simulink model "FMS"  (R2018b)
settings: configuration reference "fms_config" (kept outside this file)
values from neighbouring files (symbols this model uses):
  FMS_EXPORT = Simulink.Parameter(FMS_EXPORT_VALUE)    [fms_model_init.m]
  FMS_PARAM = Simulink.Parameter(FMS_PARAM_VALUE)    [fms_model_init.m]
undefined symbols (not defined in the file or in its folder): actuator_cmd, ax_cmd, ay_cmd, az_cmd, cmd_mask, ControlMode, ctrl_mode, DiscIntNeverNeededParam, ext_state, FMS_Cmd, FMS_CONST, home, mode, p_cmd, phi_cmd, PilotMode, psi_rate_cmd, q_cmd, r_cmd, reset, state, status, theta_cmd, throttle_cmd, timestamp, u_cmd, v_cmd, VehicleState, VehicleStatus, VTOLState, w_cmd, wp_consume, wp_current
libraries: simulink x141, FMT_Model_Lib x120, hdlsllib x13
(part 11 of 12)

== matlab function FMS/FMS Commander/Commander/Arm/MC_Mode/Auto/Mission/Mission_SubSystem/Velocity Commander/L1 Reference WP/SearchL1RefWP ==
  data: P1 input; P output; P2 input; P3 input; L1 input; u output
% Find reference waypoint (L1RefWP) on the line segment P1P2 which has 
% L1 distance from vehicle position (P3).
%
% The idea is to calculate the intersection point of a circle with L1 radius
% with the line segment P1P2.
%
% Define P = P1 + u * (P2 - P1), where P is the intersection point.
% Goal is calculating the u, where the valid u is between [0, 1].
%
% Input:
%   P1: start point of segment line
%   P2: start point of segment line
%   P3: circle center point, also is known as the vehicle position
%   L1: the L1 distance
% Output:
%   P: L1 reference waypoint
%   u: scale factor (valid between 0 and 1), -1 means no intersection.
function [P, u] = SearchL1RefWP(P1, P2, P3, L1)

% P1 = (x1, y1), P2 = (x2, y2), P3 = (x3, y3)
x1 = P1(1);
y1 = P1(2);
x2 = P2(1);
y2 = P2(2);
x3 = P3(1);
y3 = P3(2);

% The P is on circle and line segment, which yields:
A = (x2 - x1)^2 + (y2 - y1)^2;
B = 2 * ((x2 - x1)*(x1 - x3) + (y2 - y1)*(y1 - y3));
C = x3^2 + y3^2 + x1^2 + y1^2 - 2*(x3*x1 + y3*y1) - L1^2;
% Check root existence confition if B^2 - 4*A*C >= 0
D = B^2 - 4*A*C;
u = single(-1);
P = single([0 0]);

if D > 0
    % D>0 means we have 2 difference roots, % root is valid only if u is in range of [0, 1]
    u1 = (-B + sqrt(D)) / (2*A);
    u2 = (-B - sqrt(D)) / (2*A);
    
    if (u1>=0 && u1<=1) && (u2>=0 && u2<=1)
        % have 2 valid roots, select the one which is closer to P2 (target point)
        if u1 > u2
            u = u1; 
        else
            u = u2;
        end
    elseif (u1>=0 && u1<=1)
        % only 1 root valid, select it
        u = u1;
    elseif (u2>=0 && u2<=1)
        % only 1 root valid, select it
        u = u2;
    else
        % no valid root, which means no intersection point founded.
        return;
    end
elseif D == 0
    % D=0 means only 1 single root
    u1 = -B / (2*A);
    if (u1>=0 && u1<=1)
        % valid root, select it
        u = u1;
    else
        % no valid root, which means no intersection point founded.
        return;
    end
else
    % no valid root, which means no intersection point founded.
    return;
end

% calculate the L1 reference waypoint (P) coordinate
P(1) = x1 + u*(x2 - x1);
P(2) = y1 + u*(y2 - y1);

== stateflow chart FMS/FMS Commander/Commander/Arm/FW_Mode/Assist/Altitude/Altitude Command/Detect Movement/Motion Status ==
  state Hold
    entry:
    state=MotionState.Hold;
  state Move
    entry:
    state=MotionState.Move;
  state Brake
    entry:
    state=MotionState.Brake;
  (default) -> Move
  Hold -> Move : [motion_req==1]
  Move -> Brake : [motion_req==0]
  Brake -> Move [order 2] : [motion_req==1]
  Brake -> Hold [order 1] : [speed<=0.15 || after(1.5, sec)]
  data: state output Enum: MotionState; motion_req input; speed input

== stateflow chart FMS/FMS State Machine ==
  state Command_Listener [parallel]
    settings: executionOrder=1
    state Send
      entry:
      % Send command
      M.data=save_cmd;
      send(M);
    state Listen
    state Check
      entry:
      valid_cmd = CheckCmdValid(save_cmd, mode, INS_Out.flag);
    (default) -> Command_Listener.Listen
    Command_Listener.Send -> Command_Listener.Listen
    Command_Listener.Listen -> Command_Listener.Check : [hasChanged(cmd) && ...
        | cmd ~= FMS_Cmd.None]{save_cmd = cmd;}
    Command_Listener.Check -> Command_Listener.Listen [order 2]
    Command_Listener.Check -> Command_Listener.Send [order 1] : [valid_cmd == true]
  state Vehicle [parallel]
    du:
    % if mission data updated, reset waypoint index
    if hasChanged(mission_timestamp)
    wp_consume = 0;
    wp_index = 1;
    need_forwardtrans = 0;
    end
    settings: executionOrder=6
    state moved = StickMoved(stick_val,pilot_cmd) [function]
    state sp_takeoff = PrepTakeoff(xy_R) [function]
    state radius = AcceptRadius(state) [function]
    state err = HeadingErr(psi_cmd, psi_est) [function]
    state angle = WaypointAngle(start, end) [function]
    state Arm
      en:
      status = VehicleStatus.Arm;
      state SubMode
        en:
        % save enter stick value
        stick_val = [Pilot_Cmd.stick_yaw; Pilot_Cmd.stick_throttle; Pilot_Cmd.stick_roll; Pilot_Cmd.stick_pitch];
        state Return
          en:
          Cmd_In.cur_waypoint = [INS_Out.x_R; INS_Out.y_R; INS_Out.h_R];
          Cmd_In.sp_waypoint = [home(1); home(2); INS_Out.h_R]
          state Align
            en:
            Cmd_In.set_yaw = WaypointAngle(Cmd_In.cur_waypoint, Cmd_In.sp_waypoint);
            state = VehicleState.Hold;
          state Wait
          state ForwardTrans
            en:
            VTOL_M.data=VTOLMode.Fixwing;
            send(VTOL_M);
          state Execute
            en:
            state = VehicleState.Return;
          (default) -> (junction 1189)
          (junction 1189) -> Vehicle.Arm.SubMode.Return.Align [order 1] : [norm([INS_Out.x_R,INS_Out.y_R] - [home(1),home(2)]) ...
              | > 2 * AcceptRadius(VTOLState.Fixwing) && vtol_state == VTOLState.Multicopter]
          (junction 1189) -> Vehicle.Arm.SubMode.Return.Execute [order 2]
          Vehicle.Arm.SubMode.Return.Align -> Vehicle.Arm.SubMode.Return.Wait : [abs(HeadingErr(Cmd_In.set_yaw, INS_Out.psi)) <= 5/180*pi]
          Vehicle.Arm.SubMode.Return.Wait -> Vehicle.Arm.SubMode.Return.ForwardTrans : after(3, sec)
          Vehicle.Arm.SubMode.Return.ForwardTrans -> Vehicle.Arm.SubMode.Return.Execute : [vtol_state == VTOLState.ForwardTrans || ...
              | vtol_state == VTOLState.Fixwing]
        state Land
          en:
          state = VehicleState.Land;
          state MC_Land
            en:
            state = VehicleState.Land;
          state VTOL_Land
            state BackTrans
              en:
              % send BackTrans command
              VTOL_M.data=VTOLMode.Multicopter;
              send(VTOL_M);
            state Return
              en:
              Cmd_In.cur_waypoint = [INS_Out.x_R; INS_Out.y_R; INS_Out.h_R];
              Cmd_In.sp_waypoint(3) = INS_Out.h_R;
              state = VehicleState.Return;
            (default) -> Vehicle.Arm.SubMode.Land.VTOL_Land.BackTrans
            Vehicle.Arm.SubMode.Land.VTOL_Land.BackTrans -> Vehicle.Arm.SubMode.Land.VTOL_Land.Return : [vtol_state == VTOLState.Multicopter]
          Vehicle.Arm.SubMode.Land.VTOL_Land.Return -> MC_Land : [norm([INS_Out.x_R,INS_Out.y_R]-Cmd_In.sp_waypoint(1:2)') ...
              | <= AcceptRadius(vtol_state)]
          (default) -> (junction 1157)
          (junction 1157) -> Vehicle.Arm.SubMode.Land.VTOL_Land [order 2]
          (junction 1157) -> MC_Land [order 1] : [vtol_state == VTOLState.Multicopter]
        state Takeoff
          en:
          state = VehicleState.Takeoff;
        state Hold
          state BackTrans
            en:
            % If enter hold from mission, when back to mission we recover the previous vtol mode
            if state == VehicleState.Mission && ...
            (vtol_state == VTOLState.Fixwing || vtol_state == VTOLState.ForwardTrans)
            need_forwardtrans = 1;
            end
            % send BackTrans command
            VTOL_M.data=VTOLMode.Multicopter;
            send(VTOL_M);
          state Loiter
            en:
            Cmd_In.sp_waypoint = [INS_Out.x_R; INS_Out.y_R; INS_Out.h_R];
            Cmd_In.set_yaw = single(-1);
            state = VehicleState.Hold;
          (default) -> (junction 1226)
          (junction 1226) -> Vehicle.Arm.SubMode.Hold.BackTrans [order 2]
          (junction 1226) -> Vehicle.Arm.SubMode.Hold.Loiter [order 1] : [vtol_state == VTOLState.Multicopter]
          Vehicle.Arm.SubMode.Hold.BackTrans -> Vehicle.Arm.SubMode.Hold.Loiter : [vtol_state == VTOLState.Multicopter]
        Vehicle.Arm.SubMode.Takeoff -> (junction 612) : [INS_Out.h_R >= Cmd_In.sp_waypoint(3)]
        (junction 612) -> Vehicle.Arm.SubMode.Hold [order 2]
        SubMode -> Vehicle.Arm.SubMode.Hold [order 1] : M[M.data==FMS_Cmd.Pause]
        Vehicle.Arm.SubMode.Return.Execute -> Vehicle.Arm.SubMode.Land : [norm([INS_Out.x_R;INS_Out.y_R] - Cmd_In.sp_waypoint(1:2)) <= ...
            |  AcceptRadius(vtol_state)]{
            | Cmd_In.sp_waypoint = [home(1); home(2); 0]}
      state Auto
        state Offboard
          state Loiter
            en:
            state = VehicleState.Hold;
          state Run
            en:
            state = VehicleState.Offboard;
          (default) -> (junction 958)
          (junction 958) -> Vehicle.Arm.Auto.Offboard.Loiter [order 2]
          (junction 958) -> Run [order 1] : [auto_cmd_valid == 1]
          Run -> Vehicle.Arm.Auto.Offboard.Loiter : [auto_cmd_valid == 0]
          Vehicle.Arm.Auto.Offboard.Loiter -> Run : [auto_cmd_valid == 1]
        state Mission
          en:
          % Reference location of latitude and longitude, specified as an m-by-2 array, in degrees
          llo = [INS_Out.lat_0, INS_Out.lon_0] * (180/pi);
          % Set setpoint waypoint to current position
          Cmd_In.sp_waypoint = [INS_Out.x_R; INS_Out.y_R; INS_Out.h_R];
          Cmd_In.set_speed = 0;
          state pos = LLA2FLAT(lla,llo,href,psio) [function]
          state Loiter
            en:
            Cmd_In.sp_waypoint = [INS_Out.x_R; INS_Out.y_R; INS_Out.h_R];
            Cmd_In.set_yaw = single(-1);
            state = VehicleState.Hold;
          state NextWP
            en:
            if wp_index <= Mission_Data.valid_items
            nav_cmd = Mission_Data.command(wp_index);
            else
            nav_cmd = uint16(NAV_Cmd.None);
            % updated consumed waypoints
            wp_consume = wp_index - 1;
            end
          state Takeoff
            state Takeoff
              en:
              % Geodetic coordinates (latitude, longitude, and altitude), specified as an m-by-3 array in [degrees degrees meters]
              % Altitude add home(3) here because the altitude when takeoff could be non-zero
              lla = [double(Mission_Data.x(wp_index))*1e-7, double(Mission_Data.y(wp_index))*1e-7, double(-(Mission_Data.z(wp_index) + home(3)))];
              % set takeoff setpoint
              Cmd_In.sp_waypoint = LLA2FLAT(lla, llo, 0, 0);
              % enter takeoff state
              state = VehicleState.Takeoff;
            state Waypoint
              en:
              % set current waypoint to previous setpoint waypoint
              Cmd_In.cur_waypoint  = [INS_Out.x_R; INS_Out.y_R; INS_Out.h_R];
              state = VehicleState.Mission;
            (default) -> Vehicle.Arm.Auto.Mission.Takeoff.Takeoff
            Vehicle.Arm.Auto.Mission.Takeoff.Takeoff -> (junction 1270) : [INS_Out.h_R >= Cmd_In.sp_waypoint(3)]
            (junction 1270) -> (junction 1272) [order 2]
            (junction 1270) -> Vehicle.Arm.Auto.Mission.Takeoff.Waypoint [order 1] : [norm([INS_Out.x_R;INS_Out.y_R] - Cmd_In.sp_waypoint(1:2)) > ...
                |  AcceptRadius(vtol_state)]
            Vehicle.Arm.Auto.Mission.Takeoff.Waypoint -> (junction 1272) : [norm([INS_Out.x_R;INS_Out.y_R] - Cmd_In.sp_waypoint(1:2)) <= ...
                |  AcceptRadius(vtol_state)]
          state Waypoint
            en:
            % Geodetic coordinates (latitude, longitude, and altitude), specified as an m-by-3 array in [degrees degrees meters]
            % Altitude add home(3) here because the altitude when takeoff could be non-zero
            lla = [double(Mission_Data.x(wp_index))*1e-7, double(Mission_Data.y(wp_index))*1e-7, double(-(Mission_Data.z(wp_index) + home(3)))];
            % set current waypoint to previous setpoint waypoint
            Cmd_In.cur_waypoint = Cmd_In.sp_waypoint;
            % target waypoint
            Cmd_In.sp_waypoint = LLA2FLAT(lla, llo, 0, 0);
            state Align
              en:
              Cmd_In.set_yaw = WaypointAngle(Cmd_In.cur_waypoint, Cmd_In.sp_waypoint);
              state = VehicleState.Hold;
            state Hold
              en:
              Cmd_In.set_yaw = single(-1);
              state = VehicleState.Hold;
            state Wait
            state Execute
              en:
              if need_forwardtrans
              need_forwardtrans = 0;
              end
              state = VehicleState.Mission;
            state ForwardTrans
              en:
              VTOL_M.data=VTOLMode.Fixwing;
              send(VTOL_M);
            (default) -> (junction 1112)
            (junction 1112) -> Vehicle.Arm.Auto.Mission.Waypoint.Align [order 1] : [need_forwardtrans && vtol_state == VTOLState.Multicopter]
            (junction 1112) -> Vehicle.Arm.Auto.Mission.Waypoint.Execute [order 2]
            Vehicle.Arm.Auto.Mission.Waypoint.Hold -> (junction 1323) : after(Mission_Data.param1(wp_index),sec)
            Vehicle.Arm.Auto.Mission.Waypoint.Align -> Vehicle.Arm.Auto.Mission.Waypoint.Wait : [abs(HeadingErr(Cmd_In.set_yaw, INS_Out.psi)) <= 5/180*pi]
            (junction 1320) -> (junction 1323) [order 2]
            (junction 1320) -> Vehicle.Arm.Auto.Mission.Waypoint.Hold [order 1] : [Mission_Data.param1(wp_index) > 0]
            Vehicle.Arm.Auto.Mission.Waypoint.Wait -> Vehicle.Arm.Auto.Mission.Waypoint.ForwardTrans : after(2, sec)
            Vehicle.Arm.Auto.Mission.Waypoint.ForwardTrans -> Vehicle.Arm.Auto.Mission.Waypoint.Execute : [vtol_state == VTOLState.ForwardTrans || ...
                | vtol_state == VTOLState.Fixwing]
            Vehicle.Arm.Auto.Mission.Waypoint.Execute -> (junction 1320) : [norm([INS_Out.x_R;INS_Out.y_R] - Cmd_In.sp_waypoint(1:2)) <= ...
                |  AcceptRadius(vtol_state)]
          state Disarming
          state Transition
            en:
            if Mission_Data.param1(wp_index) == 3
            VTOL_M.data=VTOLMode.Multicopter;
            send(VTOL_M);
            elseif Mission_Data.param1(wp_index) == 4
            need_forwardtrans = 1;
            end
          state WaitBackTransCplt
          state Return
            en:
            % set return target pos to home
            Cmd_In.cur_waypoint = Cmd_In.sp_waypoint;
            Cmd_In.sp_waypoint = [home(1); home(2); INS_Out.h_R];
            state Align
              en:
              Cmd_In.set_yaw = WaypointAngle(Cmd_In.cur_waypoint, Cmd_In.sp_waypoint);
              state = VehicleState.Hold;
            state Wait
            state ForwardTrans
              en:
              VTOL_M.data=VTOLMode.Fixwing;
              send(VTOL_M);
            state Execute
              en:
              if need_forwardtrans
              need_forwardtrans = 0;
              end
              state = VehicleState.Return;
            (default) -> (junction 1172)
            (junction 1172) -> Vehicle.Arm.Auto.Mission.Return.Align [order 1] : [need_forwardtrans && vtol_state == VTOLState.Multicopter]
            (junction 1172) -> Vehicle.Arm.Auto.Mission.Return.Execute [order 2]
            Vehicle.Arm.Auto.Mission.Return.Align -> Vehicle.Arm.Auto.Mission.Return.Wait : [abs(HeadingErr(Cmd_In.set_yaw, INS_Out.psi)) <= 5/180*pi]
            Vehicle.Arm.Auto.Mission.Return.Wait -> Vehicle.Arm.Auto.Mission.Return.ForwardTrans : after(2, sec)
            Vehicle.Arm.Auto.Mission.Return.ForwardTrans -> Vehicle.Arm.Auto.Mission.Return.Execute : [vtol_state == VTOLState.ForwardTrans || ...
                | vtol_state == VTOLState.Fixwing]
          state VTOL_Land
            state Waypoint
              en:
              % Geodetic coordinates (latitude, longitude, and altitude), specified as an m-by-3 array in [degrees degrees meters]
              % Altitude add home(3) here because the altitude when takeoff could be non-zero
              lla = [double(Mission_Data.x(wp_index))*1e-7, double(Mission_Data.y(wp_index))*1e-7, double(-(Mission_Data.z(wp_index) + home(3)))];
              % set current waypoint to previous setpoint waypoint
              Cmd_In.cur_waypoint = Cmd_In.sp_waypoint;
              % target waypoint
              Cmd_In.sp_waypoint = LLA2FLAT(lla, llo, 0, 0);
              state Align
                en:
                Cmd_In.set_yaw = WaypointAngle(Cmd_In.cur_waypoint, Cmd_In.sp_waypoint);
                state = VehicleState.Hold;
              state Wait
              state ForwardTrans
                en:
                VTOL_M.data=VTOLMode.Fixwing;
                send(VTOL_M);
              state Execute
                en:
                if need_forwardtrans
                need_forwardtrans = 0;
                end
                state = VehicleState.Mission;
              (default) -> (junction 1282)
              (junction 1282) -> Vehicle.Arm.Auto.Mission.VTOL_Land.Waypoint.Align [order 1] : [need_forwardtrans && vtol_state == VTOLState.Multicopter]
              (junction 1282) -> Vehicle.Arm.Auto.Mission.VTOL_Land.Waypoint.Execute [order 2]
              Vehicle.Arm.Auto.Mission.VTOL_Land.Waypoint.Align -> Vehicle.Arm.Auto.Mission.VTOL_Land.Waypoint.Wait : [abs(HeadingErr(Cmd_In.set_yaw, INS_Out.psi)) <= 5/180*pi]
              Vehicle.Arm.Auto.Mission.VTOL_Land.Waypoint.Wait -> Vehicle.Arm.Auto.Mission.VTOL_Land.Waypoint.ForwardTrans : after(2, sec)
              Vehicle.Arm.Auto.Mission.VTOL_Land.Waypoint.ForwardTrans -> Vehicle.Arm.Auto.Mission.VTOL_Land.Waypoint.Execute : [vtol_state == VTOLState.ForwardTrans || ...
                  | vtol_state == VTOLState.Fixwing]
            state BackTrans
              en:
              % send BackTrans command
              VTOL_M.data=VTOLMode.Multicopter;
              send(VTOL_M);
            state Return
              en:
              Cmd_In.cur_waypoint = [INS_Out.x_R; INS_Out.y_R; INS_Out.h_R];
              % Return to land position
              if nav_cmd == NAV_Cmd.VTOL_Land || nav_cmd == NAV_Cmd.Land
              lla = [double(Mission_Data.x(wp_index))*1e-7, double(Mission_Data.y(wp_index))*1e-7, 0];
              flat = LLA2FLAT(lla, llo, 0, 0);
              Cmd_In.sp_waypoint = [flat(1); flat(2); INS_Out.h_R];
              else
              Cmd_In.sp_waypoint = [home(1); home(2); INS_Out.h_R]
              end
              state = VehicleState.Return;
            state Land
              en:
              if nav_cmd == NAV_Cmd.Land || nav_cmd == NAV_Cmd.VTOL_Land
              lla = [double(Mission_Data.x(wp_index))*1e-7, double(Mission_Data.y(wp_index))*1e-7, 0];
              Cmd_In.sp_waypoint = LLA2FLAT(lla, llo, 0, 0);
              else
              Cmd_In.sp_waypoint = [home(1); home(2); 0]
              end
              state = VehicleState.Land;
            (default) -> (junction 1278)
            (junction 1278) -> (junction 1305) [order 2]
            (junction 1278) -> Vehicle.Arm.Auto.Mission.VTOL_Land.Waypoint [order 1] : [nav_cmd == NAV_Cmd.Land || ...
                | nav_cmd == NAV_Cmd.VTOL_Land]
            (junction 1305) -> (junction 1300)
            (junction 1300) -> Vehicle.Arm.Auto.Mission.VTOL_Land.BackTrans [order 2]
            (junction 1300) -> Vehicle.Arm.Auto.Mission.VTOL_Land.Land [order 1] : [vtol_state == VTOLState.Multicopter]
            Vehicle.Arm.Auto.Mission.VTOL_Land.Waypoint.Execute -> (junction 1300) : [norm([INS_Out.x_R;INS_Out.y_R] - Cmd_In.sp_waypoint(1:2)) <= ...
                |  AcceptRadius(vtol_state)]
            Vehicle.Arm.Auto.Mission.VTOL_Land.BackTrans -> Vehicle.Arm.Auto.Mission.VTOL_Land.Return : [vtol_state == VTOLState.Multicopter]
            Vehicle.Arm.Auto.Mission.VTOL_Land.Return -> Vehicle.Arm.Auto.Mission.VTOL_Land.Land : [norm([INS_Out.x_R,INS_Out.y_R]-Cmd_In.sp_waypoint(1:2)') ...
                | <= AcceptRadius(vtol_state)]
          Mission -> NextWP : [hasChanged(mission_timestamp)]
              | {Cmd_In.set_speed = 0}
          Vehicle.Arm.Auto.Mission.VTOL_Land.Land -> (junction 1316) : [duration(on_ground) >= 2]
          (junction 1323) -> (junction 879)
          (junction 1272) -> (junction 873)
          (junction 908) -> (junction 910) : {wp_index = wp_index + 1;}
          (junction 910) -> NextWP
          (junction 873) -> (junction 908)
          (default) -> NextWP
          NextWP -> Vehicle.Arm.Auto.Mission.Takeoff [order 1] : [nav_cmd == NAV_Cmd.Takeoff && ...
              | vtol_state == VTOLState.Multicopter]
          (junction 879) -> (junction 873)
          (junction 917) -> Vehicle.Arm.Auto.Mission.Loiter [order 2]
          (junction 1119) -> Vehicle.Arm.Auto.Mission.Takeoff
          NextWP -> (junction 1119) [order 2] : [nav_cmd == NAV_Cmd.VTOL_Takeoff && ...
              | vtol_state == VTOLState.Multicopter]{need_forwardtrans = 1;}
          NextWP -> (junction 917) [order 8]
          (junction 917) -> Disarming [order 1] : [on_ground]
          NextWP -> Vehicle.Arm.Auto.Mission.Waypoint [order 3] : [nav_cmd == NAV_Cmd.Waypoint]
          (junction 1077) -> (junction 879)
          Vehicle.Arm.Auto.Mission.Return.Execute -> Vehicle.Arm.Auto.Mission.VTOL_Land : [norm([INS_Out.x_R;INS_Out.y_R] - Cmd_In.sp_waypoint(1:2)) <= ...
              |  AcceptRadius(vtol_state)]
          Transition -> (junction 1077) [order 2]
          NextWP -> Transition [order 4] : [nav_cmd == NAV_Cmd.VTOL_Transition]
          (junction 1076) -> (junction 1077)
          Transition -> WaitBackTransCplt [order 1] : [Mission_Data.param1(wp_index) == 3]
          NextWP -> (junction 1314) [order 5] : [nav_cmd == NAV_Cmd.SetSpeed]{
              | Cmd_In.set_speed = Mission_Data.param2(wp_index)}
          (junction 1314) -> (junction 1316)
          NextWP -> Vehicle.Arm.Auto.Mission.Return [order 7] : [nav_cmd == NAV_Cmd.Return]
          NextWP -> Vehicle.Arm.Auto.Mission.VTOL_Land [order 6] : [nav_cmd == NAV_Cmd.Land || ...
              | nav_cmd == NAV_Cmd.VTOL_Land]
          WaitBackTransCplt -> (junction 1076) : [vtol_state == VTOLState.Multicopter]
          (junction 915) -> (junction 1076)
          (junction 1316) -> (junction 915)
        state InvalidAutoMode
        (default) -> (junction 43)
        (junction 43) -> Offboard [order 1] : [mode == PilotMode.Offboard]
        (junction 43) -> (junction 134) [order 2]
        (junction 134) -> Mission [order 1] : [mode == PilotMode.Mission]
        (junction 134) -> InvalidAutoMode [order 2]
        Disarming -> (junction 370)
        InvalidAutoMode -> (junction 370)
      state Assist
        state InvalidAssistMode
        state Acro
          en:
          state = VehicleState.Acro;
        state Stabilize
          en:
          state = VehicleState.Stabilize;
        state Altitude
          en:
          state = VehicleState.Altitude;
        state Position
          en:
          state = VehicleState.Position;
        (default) -> (junction 354)
        (junction 354) -> (junction 190) [order 2]
        (junction 190) -> (junction 193) [order 2]
        (junction 193) -> (junction 196) [order 2]
        (junction 196) -> InvalidAssistMode [order 2]
        (junction 354) -> Acro [order 1] : [mode == PilotMode.Acro]
        (junction 190) -> Stabilize [order 1] : [mode == PilotMode.Stabilize]
        (junction 193) -> Altitude [order 1] : [mode == PilotMode.Altitude]
        (junction 196) -> Position [order 1] : [mode == PilotMode.Position]
      state Manual
        state InValidManualMode
        state Manual
          en:
          state = VehicleState.Manual;
        (default) -> (junction 410)
        (junction 410) -> InValidManualMode [order 2]
        (junction 410) -> Vehicle.Arm.Manual.Manual [order 1] : [mode == PilotMode.Manual]
      state InvalidArmMode
      Vehicle.Arm -> Vehicle.Arm.SubMode.Land [order 2] : M[M.data==FMS_Cmd.Land]
          | {Cmd_In.sp_waypoint = [INS_Out.x_R; INS_Out.y_R; 0]}
      Vehicle.Arm -> Vehicle.Arm.SubMode.Return [order 3] : M[M.data==FMS_Cmd.Return]
      Vehicle.Arm.SubMode.Hold -> Vehicle.Arm : M[M.data==FMS_Cmd.Continue ...
          | && mode ~= PilotMode.None]
      (junction 612) -> (junction 117) [order 1] : [mode ~= PilotMode.None]
      Auto -> Vehicle.Arm.SubMode.Hold : M[M.data==FMS_Cmd.Pause]
      SubMode -> (junction 117) [order 1] : [(StickMoved(stick_val, Pilot_Cmd) || ...
          | bitand(INS_Out.flag, 212) ~= 212) && ...
          | (getArmMode(mode) == 1 || getArmMode(mode) == 2)]
      Vehicle.Arm -> (junction 117) [order 1] : [hasChanged(mode) && ...
          | mode ~= PilotMode.None]
      (junction 117) -> Auto [order 1] : [getArmMode(mode) == 3]
      (default) -> (junction 117)
      (junction 117) -> (junction 140) [order 2]
      (junction 140) -> Assist [order 1] : [getArmMode(mode)  == 2]
      (junction 140) -> (junction 240) [order 2]
      (junction 240) -> Vehicle.Arm.Manual [order 1] : [getArmMode(mode)  == 1]
      (junction 240) -> InvalidArmMode [order 2]
    state Standby
      en:
      % check if mission takeoff is valid
      if mode==PilotMode.Mission
      if wp_index <= Mission_Data.valid_items > 0 && ...
      (Mission_Data.command(wp_index)==NAV_Cmd.Takeoff || ...
      Mission_Data.command(wp_index)==NAV_Cmd.VTOL_Takeoff)
      % set mission takeoff flag, so enter mission mode after 2s
      prep_mission_takeoff = 1;
      % unset prep_takeoff if prep_mission_takeoff=1
      prep_takeoff = 0;
      else
      send(DisarmEvent);
      end
      end
      % set current position as home
      home = [INS_Out.x_R; INS_Out.y_R; INS_Out.h_R; INS_Out.psi];
      % enter standby state
      state = VehicleState.Standby;
      status = VehicleStatus.Standby;
      ex:
      % on exit, unset takeoff flag
      prep_takeoff = 0;
      prep_mission_takeoff = 0;
    state Disarm
      en:
      state = VehicleState.Disarm;
      status = VehicleStatus.Disarm;
    InValidManualMode -> Vehicle
    Vehicle.Arm.SubMode.Land -> (junction 330) : [duration(on_ground) >= 2]
    (junction 330) -> Vehicle.Disarm
    (junction 332) -> (junction 334)
    (junction 334) -> Vehicle.Arm.SubMode.Takeoff : {Cmd_In.sp_waypoint = PrepTakeoff([INS_Out.x_R; INS_Out.y_R]);
        | Cmd_In.sp_waypoint(3) = Cmd_In.sp_waypoint(3) + home(3);}
    Standby -> (junction 332) [order 3] : M[M.data==FMS_Cmd.Takeoff]
    Standby -> (junction 334) [order 2] : [duration(prep_takeoff == 1) >= 2]
    (junction 989) -> Vehicle.Arm.SubMode.Hold
    (junction 987) -> (junction 989) : [pilot_cmd_lost && bitand(INS_Out.flag, 212) == 212]
    InvalidAssistMode -> Vehicle
    (junction 370) -> Vehicle
    (default) -> Vehicle.Disarm
    Assist -> (junction 987)
    Standby -> Vehicle.Disarm [order 4] : after(10, sec) || DisarmEvent
    Vehicle.Disarm -> Standby [order 1] : M[M.data==FMS_Cmd.PreArm]
    Standby -> Vehicle.Arm [order 1] : [ManualArmEvent(Pilot_Cmd) == 1 &&...
        | mode ~= PilotMode.None]
    Vehicle.Disarm -> Standby [order 2] : M[M.data==FMS_Cmd.Takeoff]
        | {prep_takeoff = 1;}
    Standby -> Vehicle.Arm [order 6] : [mode == PilotMode.Offboard && ...
        | auto_cmd_valid]
    Vehicle -> Vehicle.Disarm : M[M.data==FMS_Cmd.Disarm]
    (junction 304) -> Vehicle.Disarm
    Standby -> (junction 903) [order 5] : [duration(prep_mission_takeoff == 1) >= 2]
    (junction 903) -> Vehicle.Arm
    Vehicle.Arm -> (junction 304) [order 1] : [duration(on_ground) >= 2 && mode ~= PilotMode.Mission]
    InvalidArmMode -> Vehicle
  state Combo_Stick [parallel]
    settings: executionOrder=2
    state res = BottomRight(pilot_cmd) [function]
      (default) -> (junction 285) : {res = (pilot_cmd.stick_throttle < -0.8) && ...
          | (pilot_cmd.stick_yaw > 0.8);}
    state Idle
      du:
      bl = BottomLeft(Pilot_Cmd);
      br = BottomRight(Pilot_Cmd);
    state Arm
      en:
      M.data=FMS_Cmd.PreArm;
      send(M);
    state res = BottomLeft(pilot_cmd) [function]
      (default) -> (junction 298) : {res = (pilot_cmd.stick_throttle < -0.8) && ...
          | (pilot_cmd.stick_yaw < -0.8);}
    state Disarm
      en:
      send(DisarmEvent, Vehicle)
    (default) -> Idle
    Combo_Stick.Arm -> Idle : [~BottomRight(Pilot_Cmd)]
    Idle -> Combo_Stick.Arm [order 1] : [duration(br)>1.5]
    Idle -> Combo_Stick.Disarm [order 2] : [duration(bl)>1.5]
    Combo_Stick.Disarm -> Idle : [~BottomLeft(Pilot_Cmd)]
  state Lost_Return [parallel]
    settings: executionOrder=3
    state Lost
      en:
      % check if INS valid to return
      if bitand(INS_Out.flag, 221)
      M.data=FMS_Cmd.Return;
      send(M);
      end
    state Connect
    (default) -> Connect
    Connect -> Lost : [lost_connect]
    Lost -> Connect : [~lost_connect]
  state VTOL_Mode [parallel]
    settings: executionOrder=4
    state Send
      entry:
      % Send command
      VTOL_M.data=expect_vtol_mode;
      send(VTOL_M);
    state Listen
    state Check
      entry:
      valid_mode = CheckModeValid(expect_vtol_mode, vtol_state, INS_Out.flag);
    (default) -> VTOL_Mode.Listen
    VTOL_Mode.Send -> VTOL_Mode.Listen
    VTOL_Mode.Listen -> VTOL_Mode.Check : [hasChanged(vtol_mode)]{expect_vtol_mode = vtol_mode;}
    VTOL_Mode.Check -> VTOL_Mode.Listen [order 2]
    VTOL_Mode.Check -> VTOL_Mode.Send [order 1] : [valid_mode == true]
  state VTOL_State [parallel]
    settings: executionOrder=5
    state cplt = ForwardTransCplt(Airspeed) [function]
    state valid = IsPosValid(flag) [function]
    state res = IsStall(Airspeed) [function]
    state res = EndStall(Airspeed) [function]
    state Multicopter
      en:
      vtol_state = VTOLState.Multicopter;
    state ForwardTrans
      en:
      vtol_state = VTOLState.ForwardTrans;
    state BackwardTrans
      en:
      vtol_state = VTOLState.BackwardTrans;
    state Fixwing
      en:
      vtol_state = VTOLState.Fixwing;
    state StallProtect
      en:
      vtol_state = VTOLState.Stall;
    (default) -> Multicopter
    Multicopter -> VTOL_State.ForwardTrans : VTOL_M[VTOL_M.data==VTOLMode.Fixwing]
    BackwardTrans -> VTOL_State.ForwardTrans [order 3] : VTOL_M[VTOL_M.data==VTOLMode.Fixwing]
    BackwardTrans -> Multicopter [order 1] : [abs(Vg) < 2 || after(20, sec) || ~IsPosValid(INS_Out.flag)]
    BackwardTrans -> Multicopter [order 2] : M[M.data==FMS_Cmd.Pause]
    VTOL_State.ForwardTrans -> BackwardTrans [order 2] : VTOL_M[VTOL_M.data==VTOLMode.Multicopter]
    VTOL_State.ForwardTrans -> Fixwing [order 1] : [ForwardTransCplt(Vt)]
    Fixwing -> BackwardTrans [order 1] : VTOL_M[VTOL_M.data==VTOLMode.Multicopter]
    StallProtect -> BackwardTrans [order 1] : VTOL_M[VTOL_M.data==VTOLMode.Multicopter]
    Fixwing -> StallProtect [order 2] : [IsStall(Vt)]
    StallProtect -> Fixwing [order 2] : [EndStall(Vt)]
  data: cmd_in function_input; mode_in function_input; valid function_output; ins_flag function_input; pilotMode function_input; armMode function_output; pilot_cmd function_input; trigger function_output; stick_val function_input double size=4; moved function_output; pilot_cmd function_input Bus: Pilot_Cmd_Bus size=1; xy_R function_input single size=2; sp_takeoff function_output; radius function_output; state function_input Enum: VTOLState size=1; psi_cmd function_input single size=1; psi_est function_input single size=1; err function_output; start function_input single size=[3 1]; angle function_output; end function_input single size=[3 1]; lla function_input double size=[1 3]; llo function_input double size=[1 2]; href function_input double size=1; pos function_output; psio function_input double size=1; res function_output; pilot_cmd function_input; res function_output; pilot_cmd function_input; vtol_mode_in function_input; vtol_state_in function_input; valid function_output; ins_flag function_input; cplt function_output; Airspeed function_input single size=1; valid function_output; flag function_input uint32 size=1; res function_output; Airspeed function_input single size=1; res function_output; Airspeed function_input single size=1; state output Enum: VehicleState; vtol_state output Enum: VTOLState; cmd input; valid_cmd local; M local Enum: FMS_Cmd; mode input; Pilot_Cmd input Bus: Pilot_Cmd_Bus; lost_connect input; pilot_cmd_lost input; INS_Out input Bus: INS_Out_Bus; Mission_Data input Bus: Mission_Data_Bus; prep_takeoff local =0; stick_val local; bl local =false; br local =false; nav_cmd local uint16; wp_consume output uint8 =uint8(0); wp_index output uint8 =uint8(1); Cmd_In output Bus: Commander_In_Bus; mission_timestamp input uint32 =uint32(0); on_ground input; auto_cmd_valid input; status local Enum: VehicleStatus =VehicleStatus.None; llo local; lla local; prep_mission_takeoff local =0; save_cmd local Enum: FMS_Cmd; home data_store_memory; vtol_mode input Enum: VTOLMode; Vt input; Vg input; expect_vtol_mode local; valid_mode local; VTOL_M local Enum: VTOLMode; flat local; need_forwardtrans local
  events: DisarmEvent local FUNCTION_CALL_EVENT
  function valid = CheckCmdValid(cmd_in, mode_in, ins_flag):
    | function valid = CheckCmdValid(cmd_in, mode_in, ins_flag)
    | 
    | % bit1 |    bit2    |    bit3  |   bit4  | bit5  | bit6  |bit7|bit8|bit9
    | % init | standstill | attitude | heading | speed | LLA   | xy | h | h_AGL
    | 
    | valid = false;
    | 
    | if mode_in == PilotMode.None
    |     % Need a valid mode to handle command
    |     return;
    | end
    | 
    | % TODO: Add more checks
    | switch cmd_in
    |     case {FMS_Cmd.Takeoff, FMS_Cmd.Land, FMS_Cmd.Return, FMS_Cmd.Pause}
    |         if ~bitget(ins_flag, 1) || ~bitget(ins_flag, 3) || ~bitget(ins_flag, 4)
    |             return;
    |         end
    |         % these modes need position valid
    |         if bitget(ins_flag, 5) && bitget(ins_flag, 7) && bitget(ins_flag, 8)
    |             valid = true;
    |         end
    |     case FMS_Cmd.PreArm
    |         if ~bitget(ins_flag, 1) || ~bitget(ins_flag, 3) || ~bitget(ins_flag, 4)
    |             return;
    |         end
    |         
    |         switch mode_in
    |             case {PilotMode.Position, PilotMode.Mission, PilotMode.Offboard}
    |                 if bitget(ins_flag, 5) && bitget(ins_flag, 7) && bitget(ins_flag, 8)
    |                     valid = true;
    |                 end
    |             case PilotMode.Altitude
    |                 if bitget(ins_flag, 8)
    |                     valid = true;
    |                 end
    |             case PilotMode.Stabilize
    |                 valid = true;
    |             otherwise
    |                 % do nothing
    |         end
    |     case FMS_Cmd.Continue
    |         if mode_in == PilotMode.Offboard || mode_in == PilotMode.Mission
    |            valid = true; 
    |         end
    |     case FMS_Cmd.Disarm
    |         valid = true;   % always allowed disarm
    |     otherwise
    |         % do nothing
    | end
    | 
    | return;
  function armMode = getArmMode(pilotMode):
    | function armMode = getArmMode(pilotMode)
    | 
    | % Map pilot mode to arm mode
    | switch pilotMode
    |     case PilotMode.Manual
    |         armMode = 1;    % manual
    |     case {PilotMode.Acro, PilotMode.Stabilize, PilotMode.Altitude, PilotMode.Position}
    |         armMode = 2;    % asist
    |     case {PilotMode.Mission, PilotMode.Offboard}
    |         armMode = 3;    % auto
    |     otherwise
    |         armMode = 0;    % unknown
    | end
    | 
    | end
  function trigger = ManualArmEvent(pilot_cmd):
    | function trigger = ManualArmEvent(pilot_cmd)
    | 
    | trigger = 0;
    | 
    | % Map pilot mode to arm mode
    | switch pilot_cmd.mode
    |     case {PilotMode.Manual, PilotMode.Acro, PilotMode.Stabilize}
    |         if pilot_cmd.stick_throttle > -0.7
    |             trigger = 1;
    |         end
    |     case {PilotMode.Altitude, PilotMode.Position}
    |         if pilot_cmd.stick_throttle > 0.1
    |             trigger = 1;
    |         end
    |     otherwise
    |         % do nothing
    | end
    | 
    | end
  function valid = CheckModeValid(vtol_mode_in, vtol_state_in, ins_flag):
    | function valid = CheckModeValid(vtol_mode_in, vtol_state_in, ins_flag)
    | 
    | valid = false;
    | 
    | if (vtol_state_in == VTOLState.Multicopter || vtol_state_in == VTOLState.BackwardTrans) && vtol_mode_in == VTOLMode.Fixwing
    |     valid = true;
    | elseif (vtol_state_in == VTOLState.Fixwing || vtol_state_in == VTOLState.ForwardTrans) && vtol_mode_in == VTOLMode.Multicopter
    |     valid = true;
    | end
    | 
    | return;

== matlab function FMS/FMS Commander/Commander/Arm/MC_Mode/SubMode/Return/Velocity Commander/L1 Reference WP/OutRegionRegWP ==
  data: P1 input; P output; P2 input; P3 input
% Find the reference waypoint when vehicle is out of L1 region near P1P2.
%
% There are three region defined:
%   Region 1: The project point of P3 is lied on left side of P1P2
%   Region 2: The project point of P3 is lied on right side of P1P2
%   Region 3: The project point of P3 is lied on the segment line 
%
%   For the case of region 3, we select the project point as the reference
%   wayspoint. For the case of region 1, we choose P1 as reference waypoint
%   and similarly for the case of region 2, we choose P3 as reference
%   waypoint.
function P = OutRegionRefWP(P1, P2, P3)
% segment line P1P2
P1P2 = P2 - P1;
% segment line P1P3
P1P3 = P3 - P1;

% Define C as the P3 project point on line P1P2.
% Hence, P1C = dot(P1P3, P1P2)/|P1P2| * (P1P2/|P1P2|) = u * P1P2
% where u = dot(P1P3, P1P2) / |P1P2|^2.
u = dot(P1P3, P1P2) / sum(P1P2.^2);

if u <= 0
    % region 1
    P = P1;
elseif u >= 1
    % region 2
    P = P2;
else
    % region 3. C = P1C + P1
    P = u * P1P2 + P1;
end

== matlab function FMS/FMS Commander/Commander/Arm/MC_Mode/SubMode/Return/Velocity Commander/L1 Reference WP/SearchL1RefWP ==
  data: P1 input; P output; P2 input; P3 input; L1 input; u output
% Find reference waypoint (L1RefWP) on the line segment P1P2 which has 
% L1 distance from vehicle position (P3).
%
% The idea is to calculate the intersection point of a circle with L1 radius
% with the line segment P1P2.
%
% Define P = P1 + u * (P2 - P1), where P is the intersection point.
% Goal is calculating the u, where the valid u is between [0, 1].
%
% Input:
%   P1: start point of segment line
%   P2: start point of segment line
%   P3: circle center point, also is known as the vehicle position
%   L1: the L1 distance
% Output:
%   P: L1 reference waypoint
%   u: scale factor (valid between 0 and 1), -1 means no intersection.
function [P, u] = SearchL1RefWP(P1, P2, P3, L1)

% P1 = (x1, y1), P2 = (x2, y2), P3 = (x3, y3)
x1 = P1(1);
y1 = P1(2);
x2 = P2(1);
y2 = P2(2);
x3 = P3(1);
y3 = P3(2);

% The P is on circle and line segment, which yields:
A = (x2 - x1)^2 + (y2 - y1)^2;
B = 2 * ((x2 - x1)*(x1 - x3) + (y2 - y1)*(y1 - y3));
C = x3^2 + y3^2 + x1^2 + y1^2 - 2*(x3*x1 + y3*y1) - L1^2;
% Check root existence confition if B^2 - 4*A*C >= 0
D = B^2 - 4*A*C;
u = single(-1);
P = single([0 0]);

if D > 0
    % D>0 means we have 2 difference roots, % root is valid only if u is in range of [0, 1]
    u1 = (-B + sqrt(D)) / (2*A);
    u2 = (-B - sqrt(D)) / (2*A);
    
    if (u1>=0 && u1<=1) && (u2>=0 && u2<=1)
        % have 2 valid roots, select the one which is closer to P2 (target point)
        if u1 > u2
            u = u1; 
        else
            u = u2;
        end
    elseif (u1>=0 && u1<=1)
        % only 1 root valid, select it
        u = u1;
    elseif (u2>=0 && u2<=1)
        % only 1 root valid, select it
        u = u2;
    else
        % no valid root, which means no intersection point founded.
        return;
    end
elseif D == 0
    % D=0 means only 1 single root
    u1 = -B / (2*A);
    if (u1>=0 && u1<=1)
        % valid root, select it
        u = u1;
    else
        % no valid root, which means no intersection point founded.
        return;
    end
else
    % no valid root, which means no intersection point founded.
    return;
end

% calculate the L1 reference waypoint (P) coordinate
P(1) = x1 + u*(x2 - x1);
P(2) = y1 + u*(y2 - y1);

== stateflow chart FMS/FMS Commander/Commander/Arm/MC_Mode/SubMode/Hold/Altitude Hold/Detect Movement/Motion Status ==
  state Hold
    entry:
    state=MotionState.Hold;
  state Move
    entry:
    state=MotionState.Move;
  state Brake
    entry:
    state=MotionState.Brake;
  (default) -> Move
  Hold -> Move : [motion_req==1]
  Move -> Brake : [motion_req==0]
  Brake -> Move [order 2] : [motion_req==1]
  Brake -> Hold [order 1] : [speed<=0.15 || after(1.5, sec)]
  data: state output Enum: MotionState; motion_req input; speed input

== stateflow chart FMS/FMS Commander/Commander/Arm/MC_Mode/SubMode/Hold/Heading Hold/Detect Movement/Motion State ==
  state Hold
    entry:
    state=MotionState.Hold;
  state Move
    entry:
    state=MotionState.Move;
  state Brake
    entry:
    state=MotionState.Brake;
  (default) -> Move
  Hold -> Move : [motion_req==1]
  Move -> Brake : [motion_req==0]
  Brake -> Move [order 2] : [motion_req==1]
  Brake -> Hold [order 1] : [speed<=0.1 || after(1, sec)]
  data: state output Enum: MotionState; motion_req input; speed input

== stateflow chart FMS/FMS Commander/Commander/Arm/MC_Mode/Assist/Position/Position Command/Detect Movement/Motion State ==
  state Hold
    entry:
    state=MotionState.Hold;
  state Move
    entry:
    state=MotionState.Move;
  state Brake
    entry:
    state=MotionState.Brake;
  (default) -> Move
  Hold -> Move : [motion_req==1]
  Move -> Brake : [motion_req==0]
  Brake -> Move [order 2] : [motion_req==1]
  Brake -> Hold [order 1] : [speed<=0.2 || after(5, sec)]
  data: state output Enum: MotionState; motion_req input; speed input

== stateflow chart FMS/FMS Commander/Commander/Arm/MC_Mode/Assist/Altitude/Altitude Command/Detect Movement/Motion Status ==
  state Hold
    entry:
    state=MotionState.Hold;
  state Move
    entry:
    state=MotionState.Move;
  state Brake
    entry:
    state=MotionState.Brake;
  (default) -> Move
  Hold -> Move : [motion_req==1]
  Move -> Brake : [motion_req==0]
  Brake -> Move [order 2] : [motion_req==1]
  Brake -> Hold [order 1] : [speed<=0.15 || after(1.5, sec)]
  data: state output Enum: MotionState; motion_req input; speed input

== stateflow chart FMS/FMS Commander/Commander/Arm/MC_Mode/Assist/Altitude/Heading Command/Detect Movement/Motion State ==
  state Hold
    entry:
    state=MotionState.Hold;
  state Move
    entry:
    state=MotionState.Move;
  state Brake
    entry:
    state=MotionState.Brake;
  (default) -> Move
  Hold -> Move : [motion_req==1]
  Move -> Brake : [motion_req==0]
  Brake -> Move [order 2] : [motion_req==1]
  Brake -> Hold [order 1] : [speed<=0.1 || after(1, sec)]
  data: state output Enum: MotionState; motion_req input; speed input

== stateflow chart FMS/FMS Commander/Commander/Arm/MC_Mode/Assist/Stabilize/Heading Command/Detect Movement/Motion State ==
  state Hold
    entry:
    state=MotionState.Hold;
  state Move
    entry:
    state=MotionState.Move;
  state Brake
    entry:
    state=MotionState.Brake;
  (default) -> Move
  Hold -> Move : [motion_req==1]
  Move -> Brake : [motion_req==0]
  Brake -> Move [order 2] : [motion_req==1]
  Brake -> Hold [order 1] : [speed<=0.1 || after(1, sec)]
  data: state output Enum: MotionState; motion_req input; speed input

== stateflow chart FMS/FMS Commander/Commander/Arm/MC_Mode/Assist/Position/Altitude Command/Detect Movement/Motion Status ==
  state Hold
    entry:
    state=MotionState.Hold;
  state Move
    entry:
    state=MotionState.Move;
  state Brake
    entry:
    state=MotionState.Brake;
  (default) -> Move
  Hold -> Move : [motion_req==1]
  Move -> Brake : [motion_req==0]
  Brake -> Move [order 2] : [motion_req==1]
  Brake -> Hold [order 1] : [speed<=0.15 || after(1.5, sec)]
  data: state output Enum: MotionState; motion_req input; speed input

== stateflow chart FMS/FMS Commander/Commander/Arm/MC_Mode/Assist/Position/Heading Command/Detect Movement/Motion State ==
  state Hold
    entry:
    state=MotionState.Hold;
  state Move
    entry:
    state=MotionState.Move;
  state Brake
    entry:
    state=MotionState.Brake;
  (default) -> Move
  Hold -> Move : [motion_req==1]
  Move -> Brake : [motion_req==0]
  Brake -> Move [order 2] : [motion_req==1]
  Brake -> Hold [order 1] : [speed<=0.1 || after(1, sec)]
  data: state output Enum: MotionState; motion_req input; speed input

== stateflow chart FMS/FMS Commander/Commander/Arm/MC_Mode/SubMode/Hold/Position Hold/Detect Movement/Motion State ==
  state Hold
    entry:
    state=MotionState.Hold;
  state Move
    entry:
    state=MotionState.Move;
  state Brake
    entry:
    state=MotionState.Brake;
  (default) -> Move
  Hold -> Move : [motion_req==1]
  Move -> Brake : [motion_req==0]
  Brake -> Move [order 2] : [motion_req==1]
  Brake -> Hold [order 1] : [speed<=0.2 || after(2.5, sec)]
  data: state output Enum: MotionState; motion_req input; speed input

== stateflow chart FMS/FMS Commander/Commander/Arm/FW_Mode/Assist/Position/Altitude Command/Detect Movement/Motion Status ==
  state Hold
    entry:
    state=MotionState.Hold;
  state Move
    entry:
    state=MotionState.Move;
  state Brake
    entry:
    state=MotionState.Brake;
  (default) -> Move
  Hold -> Move : [motion_req==1]
  Move -> Brake : [motion_req==0]
  Brake -> Move [order 2] : [motion_req==1]
  Brake -> Hold [order 1] : [speed<=0.15 || after(1.5, sec)]
  data: state output Enum: MotionState; motion_req input; speed input

== matlab function FMS/FMS Commander/Commander/Arm/FW_Mode/Assist/Position/Position Command/Controller/Hold Control/L1_Reference_WP/SearchL1RefWP ==
  data: c input; P output; p0 input; n input; L1 input; t output
function [P, t] = SearchL1RefWP(c, p0, n, L1)

m = p0 - c;
A = 1;  % dot(n,n) = 1
B = 2*dot(n, m);
C = dot(m, m) - L1^2;

% Check root existence confition if B^2 - 4*A*C >= 0
D = B^2 - 4*A*C;

t = single(-1);
P = single([0;0]);

if D > 0
    % D>0 means we have 2 difference roots, % root is valid only if u is in range of [0, 1]
    u1 = (-B + sqrt(D)) / (2*A);
    u2 = (-B - sqrt(D)) / (2*A);
    
    % have 2 valid roots, select the one which is farthur
    if u1 > u2
        t = u1; 
    else
        t = u2;
    end
    
    % calculate the L1 reference waypoint (P) coordinate
    P = p0 + t*n;
elseif D == 0
    t = -B / (2*A);
    
    % calculate the L1 reference waypoint (P) coordinate
    P = p0 + t*n;
else
    % only 1 root or no valid root, use other logic to find WP.
    return;
end

== matlab function FMS/FMS Commander/Commander/Arm/FW_Mode/Assist/Position/Position Command/Controller/Hold Control/L1_Reference_WP/OutRegionRefWP ==
  data: c input; P output; p0 input; n input
function P  = OutRegionRefWP(c, p0, n)

P1P3 = c - p0;

% Define C as the P3 (vehicle) project point on ray.
% Hence, P1C = dot(P1P3, P1P2)/|P1P2| * (P1P2/|P1P2|) = t * P1P2
% where t = dot(P1P3, P1P2) / |P1P2|^2. Choose P1P2 as a normalized vector,
% therefore |P1P2| = 1, yield t = dot(P1P3, n)
t = dot(P1P3, n);
C = p0 + t*n;

% Now we calculate the distance forward from C with 30deg
d1 = norm(C - c);
d2 = d1 * tan(pi/6);

% Calculate the final waypoint
P = p0 + (t+d2)*n;

== stateflow chart FMS/FMS Commander/Commander/Arm/FW_Mode/Assist/Position/Position Command/Detect Movement/Motion State ==
  state Hold
    entry:
    state=MotionState.Hold;
  state Move
    entry:
    state=MotionState.Move;
  state Brake
    entry:
    state=MotionState.Brake;
  (default) -> Move
  Hold -> Move : [motion_req==1]
  Brake -> Move [order 2] : [motion_req==1]
  Move -> Brake : [motion_req==0]
  Brake -> Hold [order 1] : [after(2.5, sec) && speed > 5]
  data: state output Enum: MotionState; motion_req input; speed input

== matlab function FMS/FMS Commander/Commander/Arm/FW_Mode/Auto/Mission/Mission_SubSystem/Position Command/L1 Control/L1 Reference WP/NearbyRefWP ==
  data: P output; P2 input; d output; P3 input; L1 input
% Find the reference waypoint when vehicle (P3) is close to target (P2)
%
% If the vehicle is close to target (distance(P2,P3) < L1), select P2 as
% reference waypoint and return the distance, otherwise return -1.
function [P,d] = NearbyRefWP(P2, P3, L1)

P3P2 = P2 - P3;
dis = sqrt(sum(P3P2.^2));

if dis <= L1
    d = dis;
    % select P2 as reference WP
    P = P2;
else
    d = single(-1);
    % unset WP
    P = single([0; 0]);
end

== matlab function FMS/FMS Commander/Commander/Arm/FW_Mode/Auto/Mission/Mission_SubSystem/Position Command/L1 Control/L1 Reference WP/OutRegionRegWP ==
  data: P1 input; P output; P2 input; P3 input; L1 input
% Find the reference waypoint when vehicle is out of L1 region near P1P2.
%
% There are three region defined:
%   Region 1: The project point of P3 is lied on left side of P1P2
%   Region 2: The project point of P3 is lied on right side of P1P2
%   Region 3: The project point of P3 is lied on the segment line 
%
%   For the case of region 3, we select the project point as the reference
%   wayspoint. For the case of region 1, we choose P1 as reference waypoint
%   and similarly for the case of region 2, we choose P2 as reference
%   waypoint.
function P = OutRegionRefWP(P1, P2, P3, L1)
% segment line P1P2
P1P2 = P2 - P1;
% segment line P1P3
P1P3 = P3 - P1;

% Define C as the P3 project point on line P1P2.
% Hence, P1C = dot(P1P3, P1P2)/|P1P2| * (P1P2/|P1P2|) = u * P1P2
% where u = dot(P1P3, P1P2) / |P1P2|^2.
u = dot(P1P3, P1P2) / sum(P1P2.^2);

% if u <= 0
%     % region 1
%     P = P1;
% elseif u >= 1
%     % region 2
%     P = P2;
% else
%     % region 3. C = P1C + P1
%     % P = u * P1P2 + P1;
%     
%     C = u * P1P2 + P1;
%     % tan(pi/6) = 0.5774
%     u = sqrt(sum((C-P3).^2))*single(0.5774)/sqrt(sum(P1P2.^2)) + u;
%     if u > 1
%         u = single(1);
%     end
%     P = u * P1P2 + P1;
% end

if u >= 1
    % region 1: Project is on right side of P2
    P = P2;
else
    % region 2. Project is on left side of P2
    u = L1/sqrt(sum(P1P2.^2)) + u;
    
    if u > 1
        u = single(1);
    elseif u < 0
        u = single(0);
    end
    
    P = u * P1P2 + P1;
end
